simulink model "scheme_L2"  (R2025a)
settings: Solver=ode45  StartTime=0.0  StopTime=20  MaxStep=0.01  RelTol=1e-10  AbsTol=1e-12
model workspace (MAT data in the model file):
  denominators = {[1 1]; 1; [1 3 2]; [3 10 8]}
  numerators = {1; 2; 5; [2 14]}
values from neighbouring files (symbols this model uses):
  denominators = cellfun(@sym2poly, denominators, 'UniformOutput', false)    [L2.m]
  numerators = cellfun(@sym2poly, numerators, 'UniformOutput', false)    [L2.m]
settings Model: Creator=urtanto  LastModifiedBy=urtanto
settings DataIOCC: SaveFormat=Array  OutputOption=SpecifiedOutputTimes  OutputTimes=0:0.01:20

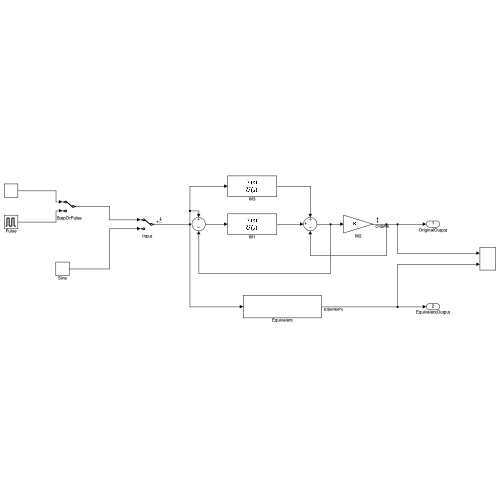
[thumbnail: Simulink's stored preview of the top-level diagram]
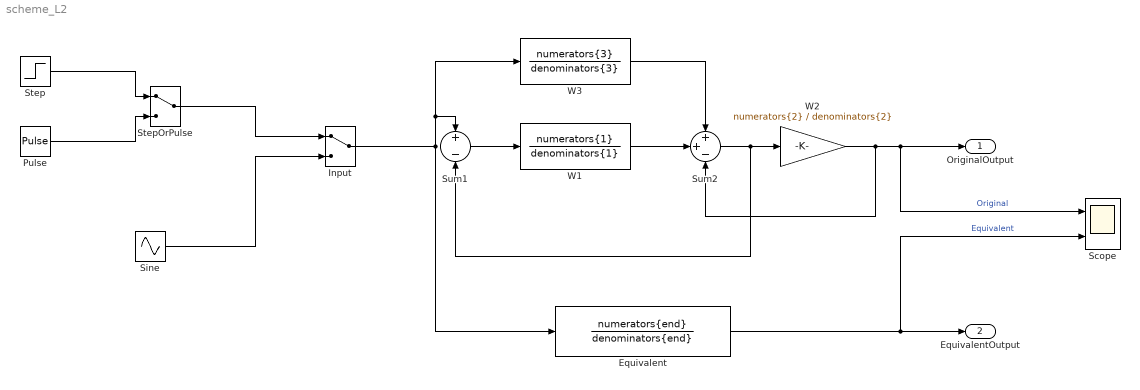
== system scheme_L2 ==
  Equivalent : TransferFcn  Numerator=numerators{end}  Denominator=denominators{end}
  Input : ManualSwitch
  Pulse : DiscretePulseGenerator  PulseType=Time based  Amplitude=10  Period=100  PulseWidth=0.1
  Scope : Scope  NumInputPorts=2
      settings: ActiveDisplayYMinimum=-1.5893671184025813  ActiveDisplayYMaximum=1.6552001605951743
  Sine : Sin  SampleTime=0
  Step : Step  Time=0  SampleTime=0
  StepOrPulse : ManualSwitch
  Sum1 : Sum  Inputs=+-
  Sum2 : Sum  Inputs=++-
  W1 : TransferFcn  Numerator=numerators{1}  Denominator=denominators{1}
  W2 : Gain  Gain=numerators{2} / denominators{2}
  W3 : TransferFcn  Numerator=numerators{3}  Denominator=denominators{3}
  OriginalOutput : Outport
  EquivalentOutput : Outport  Port=2
  wires:
  Input/1 -> Sum1/1, W3/1, Equivalent/1
  Sum1/1 -> W1/1
  W1/1 -> Sum2/2
  W3/1 -> Sum2/1
  Sum2/1 -> W2/1, Sum1/2
  W2/1 -> Scope/1, OriginalOutput/1, Sum2/3  "Original"
  Equivalent/1 -> EquivalentOutput/1, Scope/2  "Equivalent"
  Step/1 -> StepOrPulse/1
  Pulse/1 -> StepOrPulse/2
  StepOrPulse/1 -> Input/1
  Sine/1 -> Input/2
